simulink model "DIY_simuling"  (R2019a)
settings: Solver=ode23t  StartTime=0.0  StopTime=10  MaxStep=0.2  RelTol=1e-3
model workspace: external: MATLAB File D:\Users\bahaa\Desktop\gra_project\MATLAB\Assem1_DataFile.m (data not in the file)
undefined symbols (not defined in the file): ARM, J2, J3, J4, LEFT, RIGHT, Robot, smiData, TOP, X, Y, Z
libraries: sm_lib x92, nesl_utility x19
(part 3 of 3)

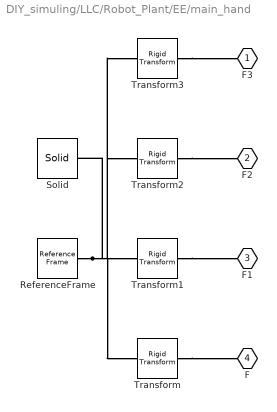
== system DIY_simuling/LLC/Robot_Plant/EE/main_hand ==
  ReferenceFrame : sm_lib/Frames and Transforms/Reference Frame
  Solid : sm_lib/Body Elements/Solid  InertiaType=Custom  Mass=smiData.Solid(10).mass  MassUnits=kg  CenterOfMass=smiData.Solid(10).CoM  CenterOfMassUnits=mm  MomentsOfInertia=smiData.Solid(10).MoI  MomentsOfInertiaUnits=kg*mm^2  ProductsOfInertia=smiData.Solid(10).PoI  ProductsOfInertiaUnits=kg*mm^2  BasedOnType=Density  Density=1000  DensityUnits=kg/m^3  DoExposeReferenceFrame=on  SerializedFrames=<Frames/>  GraphicType=FromGeometry  MarkerShape=Sphere  MarkerSize=10  GraphicVisPropType=SimpleVisualProperties  GraphicDiffuseColor=smiData.Solid(10).color  GraphicSpecularColor=[0.5 0.5 0.5 1.0]  GraphicAmbientColor=[0.15 0.15 0.15 1.0]  GraphicEmissiveColor=[0.0 0.0 0.0 1.0]  GraphicShininess=75  GraphicOpacity=smiData.Solid(10).opacity  GeometryShape=FromFile  RectangleSize=[1 1]  RectangleSizeUnits=m  BrickDimensions=[1 1 1]  BrickDimensionUnits=m  CylinderRadius=1  CylinderRadiusUnits=m  CylinderLength=1  CylinderLengthUnits=m  SphereRadius=1  SphereRadiusUnits=m  EllipsoidRadii=[1 1 1]  EllipsoidRadiiUnits=m  ExtrusionCrossSection=[1 1; -1 1; -1 -1; 1 -1]  ExtrusionCrossSectionUnits=m  ExtrusionLength=1  ExtrusionLengthUnits=m  PolygonNumSides=3  PolygonOuterRadius=1  PolygonOuterRadiusUnits=m  ExtGeomFileType=STEP  ExtGeomFileName=Robot - J5 controler.step_Default_sldprt.STEP  ExtGeomFileUnits=m  RevolutionCrossSection=[1 1; 1 -1; 2 -1; 2 1]  RevolutionCrossSectionUnits=m  RevolutionExtent=Full  RevolutionAngle=180  RevolutionAngleUnits=deg
  Transform : sm_lib/Frames and Transforms/Rigid Transform  TranslationMethod=Cartesian  TranslationStandardOffset=0  TranslationLengthUnit=mm  TranslationStandardAxis=+Z  TranslationCartesianOffset=smiData.RigidTransform(1).translation  TranslationROffset=0  TranslationROffsetUnits=m  TranslationZOffset=0  TranslationZOffsetUnits=m  TranslationThetaOffset=0  TranslationThetaOffsetUnits=deg  RotationMethod=ArbitraryAxis  RotationAngleUnits=rad  RotationStandardAxis=+Z  RotationAngle=smiData.RigidTransform(1).angle  RotationArbitraryAxis=smiData.RigidTransform(1).axis  FollAlignAxisA=+X  BaseAlignAxisA=+Y  FollAlignAxisB=+Y  BaseAlignAxisB=+Z  RotationSequenceAxes=FollowerAxes  RotationSequence=XYX  RotationSequenceAngles=[0 0 0]  RotationSequenceAnglesUnits=deg  RotationMatrix=[1 0 0; 0 1 0; 0 0 1]
  Transform1 : sm_lib/Frames and Transforms/Rigid Transform  TranslationMethod=Cartesian  TranslationStandardOffset=0  TranslationLengthUnit=mm  TranslationStandardAxis=+Z  TranslationCartesianOffset=smiData.RigidTransform(3).translation  TranslationROffset=0  TranslationROffsetUnits=m  TranslationZOffset=0  TranslationZOffsetUnits=m  TranslationThetaOffset=0  TranslationThetaOffsetUnits=deg  RotationMethod=ArbitraryAxis  RotationAngleUnits=rad  RotationStandardAxis=+Z  RotationAngle=smiData.RigidTransform(3).angle  RotationArbitraryAxis=smiData.RigidTransform(3).axis  FollAlignAxisA=+X  BaseAlignAxisA=+Y  FollAlignAxisB=+Y  BaseAlignAxisB=+Z  RotationSequenceAxes=FollowerAxes  RotationSequence=XYX  RotationSequenceAngles=[0 0 0]  RotationSequenceAnglesUnits=deg  RotationMatrix=[1 0 0; 0 1 0; 0 0 1]
  Transform2 : sm_lib/Frames and Transforms/Rigid Transform  TranslationMethod=Cartesian  TranslationStandardOffset=0  TranslationLengthUnit=mm  TranslationStandardAxis=+Z  TranslationCartesianOffset=smiData.RigidTransform(5).translation  TranslationROffset=0  TranslationROffsetUnits=m  TranslationZOffset=0  TranslationZOffsetUnits=m  TranslationThetaOffset=0  TranslationThetaOffsetUnits=deg  RotationMethod=ArbitraryAxis  RotationAngleUnits=rad  RotationStandardAxis=+Z  RotationAngle=smiData.RigidTransform(5).angle  RotationArbitraryAxis=smiData.RigidTransform(5).axis  FollAlignAxisA=+X  BaseAlignAxisA=+Y  FollAlignAxisB=+Y  BaseAlignAxisB=+Z  RotationSequenceAxes=FollowerAxes  RotationSequence=XYX  RotationSequenceAngles=[0 0 0]  RotationSequenceAnglesUnits=deg  RotationMatrix=[1 0 0; 0 1 0; 0 0 1]
  Transform3 : sm_lib/Frames and Transforms/Rigid Transform  TranslationMethod=Cartesian  TranslationStandardOffset=0  TranslationLengthUnit=mm  TranslationStandardAxis=+Z  TranslationCartesianOffset=smiData.RigidTransform(8).translation  TranslationROffset=0  TranslationROffsetUnits=m  TranslationZOffset=0  TranslationZOffsetUnits=m  TranslationThetaOffset=0  TranslationThetaOffsetUnits=deg  RotationMethod=ArbitraryAxis  RotationAngleUnits=rad  RotationStandardAxis=+Z  RotationAngle=smiData.RigidTransform(8).angle  RotationArbitraryAxis=smiData.RigidTransform(8).axis  FollAlignAxisA=+X  BaseAlignAxisA=+Y  FollAlignAxisB=+Y  BaseAlignAxisB=+Z  RotationSequenceAxes=FollowerAxes  RotationSequence=XYX  RotationSequenceAngles=[0 0 0]  RotationSequenceAnglesUnits=deg  RotationMatrix=[1 0 0; 0 1 0; 0 0 1]
  F3 : PMIOPort  Side=Left
  F2 : PMIOPort  Port=2  Side=Right
  F1 : PMIOPort  Port=3  Side=Right
  F : PMIOPort  Port=4  Side=Right
  connections:
  Solid/RConn1 -- ReferenceFrame/RConn1 -- Transform/LConn1 -- Transform1/LConn1 -- Transform2/LConn1 -- Transform3/LConn1
  Transform/RConn1 -- F/RConn1
  Transform1/RConn1 -- F1/RConn1
  Transform2/RConn1 -- F2/RConn1
  Transform3/RConn1 -- F3/RConn1

== system DIY_simuling/LLC/Robot_Plant/EE/scrow ==
  ReferenceFrame : sm_lib/Frames and Transforms/Reference Frame
  Solid : sm_lib/Body Elements/Solid  InertiaType=Custom  Mass=smiData.Solid(9).mass  MassUnits=kg  CenterOfMass=smiData.Solid(9).CoM  CenterOfMassUnits=mm  MomentsOfInertia=smiData.Solid(9).MoI  MomentsOfInertiaUnits=kg*mm^2  ProductsOfInertia=smiData.Solid(9).PoI  ProductsOfInertiaUnits=kg*mm^2  BasedOnType=Density  Density=1000  DensityUnits=kg/m^3  DoExposeReferenceFrame=on  SerializedFrames=<Frames/>  GraphicType=FromGeometry  MarkerShape=Sphere  MarkerSize=10  GraphicVisPropType=SimpleVisualProperties  GraphicDiffuseColor=smiData.Solid(9).color  GraphicSpecularColor=[0.5 0.5 0.5 1.0]  GraphicAmbientColor=[0.15 0.15 0.15 1.0]  GraphicEmissiveColor=[0.0 0.0 0.0 1.0]  GraphicShininess=75  GraphicOpacity=smiData.Solid(9).opacity  GeometryShape=FromFile  RectangleSize=[1 1]  RectangleSizeUnits=m  BrickDimensions=[1 1 1]  BrickDimensionUnits=m  CylinderRadius=1  CylinderRadiusUnits=m  CylinderLength=1  CylinderLengthUnits=m  SphereRadius=1  SphereRadiusUnits=m  EllipsoidRadii=[1 1 1]  EllipsoidRadiiUnits=m  ExtrusionCrossSection=[1 1; -1 1; -1 -1; 1 -1]  ExtrusionCrossSectionUnits=m  ExtrusionLength=1  ExtrusionLengthUnits=m  PolygonNumSides=3  PolygonOuterRadius=1  PolygonOuterRadiusUnits=m  ExtGeomFileType=STEP  ExtGeomFileName=Robot - J7 thread.step_Default_sldprt.STEP  ExtGeomFileUnits=m  RevolutionCrossSection=[1 1; 1 -1; 2 -1; 2 1]  RevolutionCrossSectionUnits=m  RevolutionExtent=Full  RevolutionAngle=180  RevolutionAngleUnits=deg
  Transform : sm_lib/Frames and Transforms/Rigid Transform  TranslationMethod=Cartesian  TranslationStandardOffset=0  TranslationLengthUnit=mm  TranslationStandardAxis=+Z  TranslationCartesianOffset=smiData.RigidTransform(4).translation  TranslationROffset=0  TranslationROffsetUnits=m  TranslationZOffset=0  TranslationZOffsetUnits=m  TranslationThetaOffset=0  TranslationThetaOffsetUnits=deg  RotationMethod=ArbitraryAxis  RotationAngleUnits=rad  RotationStandardAxis=+Z  RotationAngle=smiData.RigidTransform(4).angle  RotationArbitraryAxis=smiData.RigidTransform(4).axis  FollAlignAxisA=+X  BaseAlignAxisA=+Y  FollAlignAxisB=+Y  BaseAlignAxisB=+Z  RotationSequenceAxes=FollowerAxes  RotationSequence=XYX  RotationSequenceAngles=[0 0 0]  RotationSequenceAnglesUnits=deg  RotationMatrix=[1 0 0; 0 1 0; 0 0 1]
  F : PMIOPort  Side=Left
  connections:
  Solid/RConn1 -- ReferenceFrame/RConn1 -- Transform/LConn1
  Transform/RConn1 -- F/RConn1

== matlab function DIY_simuling/LLC/Linear Joint Reference Model/MATLAB Function ==
  data: x6_ref input; xm6dot output; xm6 input; x6_m output; dx6_m output; ddx6_m output
function [xm6dot, x6_m, dx6_m, ddx6_m] = Linear_Reference_Model(x6_ref, xm6)

% =========================================================
% Second-order reference model for linear joint x6
% Range: 0 <= x6 <= 0.022 m
% =========================================================

% Force scalar reference
x6_ref = min(max(x6_ref, 0), 0.022);

% State vector
xm6 = reshape(xm6, [2,1]);

% Parameters
zeta = 1;
wn   = 2;

% State-space model
A = [
    0, 1;
   -wn^2, -2*zeta*wn
];

B = [
    0;
    wn^2
];

% Dynamics
xm6dot = A*xm6 + B*x6_ref;

% Outputs
x6_m   = xm6(1);
dx6_m  = xm6(2);
ddx6_m = xm6dot(2);

end

== matlab function DIY_simuling/LLC/Refrense model/MATLAB Function ==
  data: qref input; xmdot output; xm input; qm output; dqm output; ddqm output
function [xmdot, qm, dqm, ddqm] = Reference_Model_Law(qref, xm)

% =========================================================
% Second-order reference model
% qref -> qm, dqm, ddqm
% =========================================================

qref = reshape(qref, [5,1]);
xm   = reshape(xm,   [10,1]);

% Predefine outputs
xmdot = zeros(10,1);
qm    = zeros(5,1);
dqm   = zeros(5,1);
ddqm  = zeros(5,1);

% Reference model parameters
zeta = [1; 1; 1; 1; 1];
wn   = [2; 2; 2; 2; 2];

Z = diag(zeta);
Omega = diag(wn);

Am = [
    zeros(5,5), eye(5);
    -Omega^2,  -2*Z*Omega
];

Bm = [
    zeros(5,5);
    Omega^2
];

% Reference model dynamics
xmdot = Am*xm + Bm*qref;

% Outputs
qm   = xm(1:5);
dqm  = xm(6:10);
ddqm = xmdot(6:10);

end

== matlab function DIY_simuling/MATLAB Function ==
  data: x_cm input; q1_ref output; y_cm input; z_cm input; q2_ref output; q3_ref output; q4_ref output; q5_ref output
function [q1_ref, q2_ref, q3_ref, q4_ref, q5_ref] = IK_Block(x_cm, y_cm, z_cm)

% =========================================================
% IK Block for Simulink
%
% Inputs:
% x_cm, y_cm, z_cm : desired end-effector position [cm]
%
% Outputs:
% q1_ref ... q5_ref : joint reference angles [rad]
%
% Notes:
% - Uses DH-based Generalized IK from base workspace.
% - IK solves DH total angles.
% - theta_offset_DH is subtracted to get real joint angles.
% =========================================================

coder.extrinsic('assignin');
coder.extrinsic('evalin');

% -----------------------------
% Initialize scalar outputs
% -----------------------------
q1_ref = 0;
q2_ref = 0;
q3_ref = 0;
q4_ref = 0;
q5_ref = 0;

% -----------------------------
% Send desired position to base workspace
% -----------------------------
assignin('base', 'ik_x_cm', x_cm);
assignin('base', 'ik_y_cm',-1*y_cm);
assignin('base', 'ik_z_cm', z_cm);

% -----------------------------
% Run IK in base workspace
% -----------------------------
evalin('base', [ ...
    'posTarget_DH.TargetPosition = [ik_x_cm ik_y_cm ik_z_cm] / 100;' ...
    '[qSol_IK, solInfo_IK] = gik_DH(q_prev_IK, posTarget_DH);' ...
    'q_prev_IK = qSol_IK;' ...
    'q_out_IK = qSol_IK - theta_offset_DH;' ...
]);

% -----------------------------
% Read IK result
% q_out_IK is in rad
% -----------------------------
q_tmp = evalin('base', 'q_out_IK');

% -----------------------------
% Separate outputs
% -----------------------------
q1_ref = q_tmp(1);
q2_ref = q_tmp(2);
q3_ref = q_tmp(3);
q4_ref = q_tmp(4);
q5_ref = q_tmp(5);

end

== matlab function DIY_simuling/MATLAB Function1 ==
  data: q1 input; x_cm output; q2 input; q3 input; q4 input; q5 input; y_cm output; z_cm output
function [x_cm, y_cm, z_cm] = FK_xyz(q1, q2, q3, q4, q5)

% =========================================================
% Forward Kinematics for 5-DOF robotic arm
%
% Inputs:
% q1..q5 : joint angles [rad]
%
% Outputs:
% x_cm, y_cm, z_cm : end-effector position [cm]
% =========================================================

q = [
    q1;
    q2;
    q3;
    q4;
    q5
];

% -----------------------------
% Robot dimensions [m]
% -----------------------------
a1 = 0.017;
l1 = 0.05;
l2 = 0.12;
l3 = 0.044;
l4 = 0.15;
l5 = 0.152;

% -----------------------------
% Forward kinematics
% Standard DH:
% A = RotZ(theta)*TransZ(d)*TransX(a)*RotX(alpha)
% -----------------------------
T = eye(4);

T = T * DH(a1,  pi/2, l1, q(1));
T = T * DH(l2,  0,    0,  q(2) + pi/2);
T = T * DH(l3,  pi/2, 0,  q(3));
T = T * DH(0,   pi/2, l4, q(4) + pi);
T = T * DH(l5,  0,    0,  q(5) + pi/2);

% Position in meters
p = T(1:3,4);

% Convert to cm
x_cm = p(1) * 100;
y_cm = p(2) * 100;
z_cm = p(3) * 100;

end


% =========================================================
% DH transformation
% =========================================================
function A = DH(a, alpha, d, theta)

ct = cos(theta);
st = sin(theta);
ca = cos(alpha);
sa = sin(alpha);

A = [
    ct, -st*ca,  st*sa, a*ct;
    st,  ct*ca, -ct*sa, a*st;
    0,      sa,     ca,    d;
    0,       0,      0,    1
];

end

== matlab function DIY_simuling/MATLAB Function2 ==
  data: ex input; dx output; ey input; ez input; dy output; dz output
function [dx, dy, dz] = Controller(ex, ey, ez)

dx = 0;
dy = 0;
dz = 0;

end

== matlab function DIY_simuling/MATLAB Function3 ==
  data: x_ref input; q6_cmd output; y_ref input; z_ref input; x_act input; y_act input; z_act input
function q6_cmd = Close_Fingers_Command(x_ref, y_ref, z_ref, x_act, y_act, z_act)

% Error in cm
ex = x_ref - x_act;
ey = y_ref - y_act;
ez = z_ref - z_act;

e_norm = sqrt(ex^2 + ey^2 + ez^2);

% reaching tolerance [cm]
tol_cm = 0.5;

if e_norm < tol_cm
    q6_cmd = 0.022;   % close
else
    q6_cmd = 0;       % open
end

end
